simulink model "Bossi_Emanuele_EE460S3D_R99"  (R2025a)
settings: Solver=FixedStepDiscrete  StartTime=0.0  StopTime=120  FixedStep=dt0  RelTol=1e-3  EnableMultiTasking=on
PostLoadFcn:
  | %Set the size for the model
  | set_param(gcs,'Location',[10 10 1270 970])
  | %Set the zoom factor for the model
  | set_param(gcs,'ZoomFactor','100')
InitFcn:
  | tic
  | Bossi_Emanuele_EE460_Final
  | INIT_S3D_01
StartFcn:
  | tend0=toc;
  | tic;
StopFcn:
  | tend=toc;
  | disp(['Simulation time = ' num2str(tout(end)) ' sec'])
  | disp(['Real time = ' num2str(tend) ' sec'])
  | title('DONE')
  | SCORE=round((max(0,120-tout(end)-tend0))*4+10*(40-FuelBurned)+sum(100*double(PDONE)-100*double(PDONE<.5)));
  | PlotS3D(PlotInput);
  | text(15,22,['S: ' num2str(SCORE)]);
  | % Reset color scheme back to normal defaults
  | figure()
  | blkwhitebg('w');
  | close
values from neighbouring files (symbols this model uses):
  A_obs = [ 0  1  0  0  0  0 ... (first row only)    [Bossi_Emanuele_EE460_Final.m]
  B_obs = [ 0     0     0 ... (first row only)    [Bossi_Emanuele_EE460_Final.m]
  C_obs = [ 1 0 0 0 0 0 ... (first row only)    [Bossi_Emanuele_EE460_Final.m]
  d2r = pi/180    (= 0.0174532925199)    [INIT_S3D_01.m]
  D_obs = [ 0     0     0 ... (first row only)    [Bossi_Emanuele_EE460_Final.m]
  dt = 0.01    [INIT_S3D_01.m]
  dt0 = 0.001    [INIT_S3D_01.m]
  fr = 100    [INIT_S3D_01.m]
  G = [1,  1, -1, -1,  0,  0,  0,  0 ... (first row only)    [Bossi_Emanuele_EE460_Final.m]
  G_obs = eye(6)    [Bossi_Emanuele_EE460_Final.m]
  HM_S = 250    [INIT_S3D_01.m]
  HM_U = 500    [INIT_S3D_01.m]
  J = Jbase+JC0+JF+M*(Xcg^2+Ycg^2)    [INIT_S3D_01.m]
  Jbase = JC1+4*Ja+2*Ma*da^2+2*Ma*db^2    [INIT_S3D_01.m]
  JC0 = MC0/2    (= 10.2101761242)    [INIT_S3D_01.m]
  Kdtheta = 2 * zeta_th * wn_th * J_eff    [Bossi_Emanuele_EE460_Final.m]
  Kdtheta_fail = 2 * zeta_th_fail * wn_th_fail * J_eff    [Bossi_Emanuele_EE460_Final.m]
  Kdx = 2 * zeta_xy * wn_xy * M_eff    [Bossi_Emanuele_EE460_Final.m]
  Kdx_fail = 2 * zeta_xy_fail * wn_xy_fail * M_eff    [Bossi_Emanuele_EE460_Final.m]
  Kdy = 2 * zeta_xy * wn_xy * M_eff    [Bossi_Emanuele_EE460_Final.m]
  Kdy_fail = 2 * zeta_xy_fail * wn_xy_fail * M_eff    [Bossi_Emanuele_EE460_Final.m]
  Kptheta = J_eff * wn_th^2    [Bossi_Emanuele_EE460_Final.m]
  Kptheta_fail = J_eff * wn_th_fail^2    [Bossi_Emanuele_EE460_Final.m]
  Kpx = M_eff * wn_xy^2    [Bossi_Emanuele_EE460_Final.m]
  Kpx_fail = M_eff * wn_xy_fail^2    [Bossi_Emanuele_EE460_Final.m]
  Kpy = M_eff * wn_xy^2    [Bossi_Emanuele_EE460_Final.m]
  Kpy_fail = M_eff * wn_xy_fail^2    [Bossi_Emanuele_EE460_Final.m]
  L13 = sqrt(10)    [INIT_S3D_01.m]
  L24 = sqrt(6.25)    [INIT_S3D_01.m]
  LVL = LVL12    [INIT_S3D_01.m]
  M = MC+M1+M2+M3+M4+4*Ma    [INIT_S3D_01.m]
  M1 = LVL.M1    [INIT_S3D_01.m]
  M2 = LVL.M2    [INIT_S3D_01.m]
  M3 = LVL.M3    [INIT_S3D_01.m]
  M4 = LVL.M4    [INIT_S3D_01.m]
  max_qddot = [max_qddot_x; max_qddot_y; max_qddot_theta]    [Bossi_Emanuele_EE460_Final.m]
  mdti = (1/300)    (= 0.00333333333333)    [INIT_S3D_01.m]
  P = [1  1 -1 -1  0  0  0  0 ... (first row only)    [Bossi_Emanuele_EE460_Final.m]
  Pdata = [LVL.P1 LVL.P2 LVL.P3 LVL.P4]    [INIT_S3D_01.m]    (also in PlotS3D.m = R*[xt1;yt1+[0 3*tt*TV(idx-13)*TSIG(idx-13) 0]])
  PTvec = [Pdata(:,1);Pdata(:,2);Pdata(:,3);Pdata(:,4) ... (first row only)    [INIT_S3D_01.m]
  Q_obs = eye(6)    [Bossi_Emanuele_EE460_Final.m]
  r2d = 180/pi    (= 57.2957795131)    [INIT_S3D_01.m]
  r_bang = 0.5    [Bossi_Emanuele_EE460_Final.m]
  Sconfig = 1    [Bossi_Emanuele_EE460_Final.m]
  SLIM = [-100 100 ... (first row only)    [INIT_S3D_01.m]
  SQ = [.005 .01 .004 .005 .01 .004 .02 .01 .4]'    [INIT_S3D_01.m]
  SSF = 1./SQ    [INIT_S3D_01.m]
  tau = 0.5    [Bossi_Emanuele_EE460_Final.m]
  TOLdata = [LVL.P1tol LVL.P2tol LVL.P3tol LVL.P4tol]    [INIT_S3D_01.m]
  ULIM = [[Umin Umax];0 0;0 0]    [INIT_S3D_01.m]
undefined symbols (not defined in the file or in its folder): den_lp, den_lp2, DiscIntNeverNeededParam, dt1_bang_3, dt2_bang_3, dtc_bang_3, num_lp, num_lp2, q0_1
libraries: simulink x87, matrix_library x4, sl3dlib x1, aerolibutil x1, aerolibanimutils x1
(part 6 of 8)

== system Bossi_Emanuele_EE460S3D_R99/S3D_Plant/ThrusterValues/FailModes/Ufail4 ==
  Uin : Inport
  MP : Inport  Port=2
  Bus Selector1 : BusSelector  OutputSignals=U1cmd,U2cmd,U3cmd,U4cmd,U5cmd,U6cmd,U7cmd,U8cmd,U9cmd,U10cmd  OutputAsBus=on
  Bus Selector2 : BusSelector  OutputSignals=MfuelVector
  Bus to Vector2 : BusToVector
  CURRENT : Subsystem  TreatAsAtomicUnit=on
  Compare To Constant2 : simulink/Logic and Bit Operations/Compare To Constant  relop=>  const=eps  OutDataTypeStr=boolean
  Constant2 : Constant  Value=LVL.Uft(Udx,1)+rand*(LVL.Uft(Udx,2)-LVL.Uft(Udx,1))  SampleTime=dt0
  Constant3 : Constant  Value=LVL.Ufail(Udx)  SampleTime=dt0
  Constant4 : Constant  Value=-1  SampleTime=dt0
  Digital Clock : DigitalClock  SampleTime=dt0
  FailLogic : Subsystem
  If : If  IfExpression=u1 < -0.5  ElseIfExpressions=u1 > 0.5 & u1 < 1.5  SampleTime=dt0
  MAX : Subsystem  TreatAsAtomicUnit=on
  MIN : Subsystem  TreatAsAtomicUnit=on
  Merge : Merge  Inputs=3
  Relational Operator : RelationalOperator  Operator=<  OutDataTypeStr=boolean  InputSameDT=off
  Selector1 : Selector  InputPortWidth=4  IndexOptions=Index vector (dialog)  Indices=[Tank]  OutputSizes=1
  Selector2 : Selector  InputPortWidth=10  IndexOptions=Index vector (dialog)  Indices=[Udx]  OutputSizes=1
  Switch : Switch  Criteria=u2 > Threshold  SaturateOnIntegerOverflow=off  InputSameDT=off
  Switch1 : Switch  Criteria=u2 > Threshold  SaturateOnIntegerOverflow=off  InputSameDT=off
  Unit Delay : UnitDelay  SampleTime=dt0  HasFrameUpgradeWarning=on
  Uout : Outport
  wires:
  Selector2/1 -> Switch/1
  Bus to Vector2/1 -> Selector2/1
  Bus Selector1/1 -> Bus to Vector2/1
  FailLogic/1(NoFail) -> Switch/2
  Compare To Constant2/1 -> Switch1/2, FailLogic/2(FuelRemaining)
  Relational Operator/1 -> FailLogic/1(BeforeFail)
  Constant4/1 -> Switch1/3
  Constant3/1 -> Switch1/1
  Selector1/1 -> Compare To Constant2/1
  Bus Selector2/1 -> Selector1/1  "<MfuelVector>"
  MP/1 -> Bus Selector2/1
  Switch/1 -> Unit Delay/1, Uout/1
  Switch1/1 -> If/1, FailLogic/3(FailMode)
  Uin/1 -> Bus Selector1/1
  Merge/1 -> Switch/3
  MIN/1(Out1) -> Merge/1
  CURRENT/1(Out1) -> Merge/3
  Constant2/1 -> Relational Operator/2
  MAX/1(Out1) -> Merge/2
  Unit Delay/1 -> CURRENT/1(In1)
  If/3 -> CURRENT/Action
  Digital Clock/1 -> Relational Operator/1
  If/2 -> MAX/Action
  If/1 -> MIN/Action

== system Bossi_Emanuele_EE460S3D_R99/S3D_Plant/ThrusterValues/FailModes/Ufail5 ==
  Uin : Inport
  MP : Inport  Port=2
  Bus Selector1 : BusSelector  OutputSignals=U1cmd,U2cmd,U3cmd,U4cmd,U5cmd,U6cmd,U7cmd,U8cmd,U9cmd,U10cmd  OutputAsBus=on
  Bus Selector2 : BusSelector  OutputSignals=MfuelVector
  Bus to Vector2 : BusToVector
  CURRENT : Subsystem  TreatAsAtomicUnit=on
  Compare To Constant2 : simulink/Logic and Bit Operations/Compare To Constant  relop=>  const=eps  OutDataTypeStr=boolean
  Constant2 : Constant  Value=LVL.Uft(Udx,1)+rand*(LVL.Uft(Udx,2)-LVL.Uft(Udx,1))  SampleTime=dt0
  Constant3 : Constant  Value=LVL.Ufail(Udx)  SampleTime=dt0
  Constant4 : Constant  Value=-1  SampleTime=dt0
  Digital Clock : DigitalClock  SampleTime=dt0
  FailLogic : Subsystem
  If : If  IfExpression=u1 < -0.5  ElseIfExpressions=u1 > 0.5 & u1 < 1.5  SampleTime=dt0
  MAX : Subsystem  TreatAsAtomicUnit=on
  MIN : Subsystem  TreatAsAtomicUnit=on
  Merge : Merge  Inputs=3
  Relational Operator : RelationalOperator  Operator=<  OutDataTypeStr=boolean  InputSameDT=off
  Selector1 : Selector  InputPortWidth=4  IndexOptions=Index vector (dialog)  Indices=[Tank]  OutputSizes=1
  Selector2 : Selector  InputPortWidth=10  IndexOptions=Index vector (dialog)  Indices=[Udx]  OutputSizes=1
  Switch : Switch  Criteria=u2 > Threshold  SaturateOnIntegerOverflow=off  InputSameDT=off
  Switch1 : Switch  Criteria=u2 > Threshold  SaturateOnIntegerOverflow=off  InputSameDT=off
  Unit Delay : UnitDelay  SampleTime=dt0  HasFrameUpgradeWarning=on
  Uout : Outport
  wires:
  Selector2/1 -> Switch/1
  Bus to Vector2/1 -> Selector2/1
  Bus Selector1/1 -> Bus to Vector2/1
  FailLogic/1(NoFail) -> Switch/2
  Compare To Constant2/1 -> Switch1/2, FailLogic/2(FuelRemaining)
  Relational Operator/1 -> FailLogic/1(BeforeFail)
  Constant4/1 -> Switch1/3
  Constant3/1 -> Switch1/1
  Selector1/1 -> Compare To Constant2/1
  Bus Selector2/1 -> Selector1/1  "<MfuelVector>"
  MP/1 -> Bus Selector2/1
  Switch/1 -> Unit Delay/1, Uout/1
  Switch1/1 -> If/1, FailLogic/3(FailMode)
  Uin/1 -> Bus Selector1/1
  Merge/1 -> Switch/3
  MIN/1(Out1) -> Merge/1
  CURRENT/1(Out1) -> Merge/3
  Constant2/1 -> Relational Operator/2
  MAX/1(Out1) -> Merge/2
  Unit Delay/1 -> CURRENT/1(In1)
  If/3 -> CURRENT/Action
  Digital Clock/1 -> Relational Operator/1
  If/2 -> MAX/Action
  If/1 -> MIN/Action

== system Bossi_Emanuele_EE460S3D_R99/S3D_Plant/ThrusterValues/FailModes/Ufail6 ==
  Uin : Inport
  MP : Inport  Port=2
  Bus Selector1 : BusSelector  OutputSignals=U1cmd,U2cmd,U3cmd,U4cmd,U5cmd,U6cmd,U7cmd,U8cmd,U9cmd,U10cmd  OutputAsBus=on
  Bus Selector2 : BusSelector  OutputSignals=MfuelVector
  Bus to Vector2 : BusToVector
  CURRENT : Subsystem  TreatAsAtomicUnit=on
  Compare To Constant2 : simulink/Logic and Bit Operations/Compare To Constant  relop=>  const=eps  OutDataTypeStr=boolean
  Constant2 : Constant  Value=LVL.Uft(Udx,1)+rand*(LVL.Uft(Udx,2)-LVL.Uft(Udx,1))  SampleTime=dt0
  Constant3 : Constant  Value=LVL.Ufail(Udx)  SampleTime=dt0
  Constant4 : Constant  Value=-1  SampleTime=dt0
  Digital Clock : DigitalClock  SampleTime=dt0
  FailLogic : Subsystem
  If : If  IfExpression=u1 < -0.5  ElseIfExpressions=u1 > 0.5 & u1 < 1.5  SampleTime=dt0
  MAX : Subsystem  TreatAsAtomicUnit=on
  MIN : Subsystem  TreatAsAtomicUnit=on
  Merge : Merge  Inputs=3
  Relational Operator : RelationalOperator  Operator=<  OutDataTypeStr=boolean  InputSameDT=off
  Selector1 : Selector  InputPortWidth=4  IndexOptions=Index vector (dialog)  Indices=[Tank]  OutputSizes=1
  Selector2 : Selector  InputPortWidth=10  IndexOptions=Index vector (dialog)  Indices=[Udx]  OutputSizes=1
  Switch : Switch  Criteria=u2 > Threshold  SaturateOnIntegerOverflow=off  InputSameDT=off
  Switch1 : Switch  Criteria=u2 > Threshold  SaturateOnIntegerOverflow=off  InputSameDT=off
  Unit Delay : UnitDelay  SampleTime=dt0  HasFrameUpgradeWarning=on
  Uout : Outport
  wires:
  Selector2/1 -> Switch/1
  Bus to Vector2/1 -> Selector2/1
  Bus Selector1/1 -> Bus to Vector2/1
  FailLogic/1(NoFail) -> Switch/2
  Compare To Constant2/1 -> Switch1/2, FailLogic/2(FuelRemaining)
  Relational Operator/1 -> FailLogic/1(BeforeFail)
  Constant4/1 -> Switch1/3
  Constant3/1 -> Switch1/1
  Selector1/1 -> Compare To Constant2/1
  Bus Selector2/1 -> Selector1/1  "<MfuelVector>"
  MP/1 -> Bus Selector2/1
  Switch/1 -> Unit Delay/1, Uout/1
  Switch1/1 -> If/1, FailLogic/3(FailMode)
  Uin/1 -> Bus Selector1/1
  Merge/1 -> Switch/3
  MIN/1(Out1) -> Merge/1
  CURRENT/1(Out1) -> Merge/3
  Constant2/1 -> Relational Operator/2
  MAX/1(Out1) -> Merge/2
  Unit Delay/1 -> CURRENT/1(In1)
  If/3 -> CURRENT/Action
  Digital Clock/1 -> Relational Operator/1
  If/2 -> MAX/Action
  If/1 -> MIN/Action

== system Bossi_Emanuele_EE460S3D_R99/S3D_Plant/ThrusterValues/FailModes/Ufail7 ==
  Uin : Inport
  MP : Inport  Port=2
  Bus Selector1 : BusSelector  OutputSignals=U1cmd,U2cmd,U3cmd,U4cmd,U5cmd,U6cmd,U7cmd,U8cmd,U9cmd,U10cmd  OutputAsBus=on
  Bus Selector2 : BusSelector  OutputSignals=MfuelVector
  Bus to Vector2 : BusToVector
  CURRENT : Subsystem  TreatAsAtomicUnit=on
  Compare To Constant2 : simulink/Logic and Bit Operations/Compare To Constant  relop=>  const=eps  OutDataTypeStr=boolean
  Constant2 : Constant  Value=LVL.Uft(Udx,1)+rand*(LVL.Uft(Udx,2)-LVL.Uft(Udx,1))  SampleTime=dt0
  Constant3 : Constant  Value=LVL.Ufail(Udx)  SampleTime=dt0
  Constant4 : Constant  Value=-1  SampleTime=dt0
  Digital Clock : DigitalClock  SampleTime=dt0
  FailLogic : Subsystem
  If : If  IfExpression=u1 < -0.5  ElseIfExpressions=u1 > 0.5 & u1 < 1.5  SampleTime=dt0
  MAX : Subsystem  TreatAsAtomicUnit=on
  MIN : Subsystem  TreatAsAtomicUnit=on
  Merge : Merge  Inputs=3
  Relational Operator : RelationalOperator  Operator=<  OutDataTypeStr=boolean  InputSameDT=off
  Selector1 : Selector  InputPortWidth=4  IndexOptions=Index vector (dialog)  Indices=[Tank]  OutputSizes=1
  Selector2 : Selector  InputPortWidth=10  IndexOptions=Index vector (dialog)  Indices=[Udx]  OutputSizes=1
  Switch : Switch  Criteria=u2 > Threshold  SaturateOnIntegerOverflow=off  InputSameDT=off
  Switch1 : Switch  Criteria=u2 > Threshold  SaturateOnIntegerOverflow=off  InputSameDT=off
  Unit Delay : UnitDelay  SampleTime=dt0  HasFrameUpgradeWarning=on
  Uout : Outport
  wires:
  Selector2/1 -> Switch/1
  Bus to Vector2/1 -> Selector2/1
  Bus Selector1/1 -> Bus to Vector2/1
  FailLogic/1(NoFail) -> Switch/2
  Compare To Constant2/1 -> Switch1/2, FailLogic/2(FuelRemaining)
  Relational Operator/1 -> FailLogic/1(BeforeFail)
  Constant4/1 -> Switch1/3
  Constant3/1 -> Switch1/1
  Selector1/1 -> Compare To Constant2/1
  Bus Selector2/1 -> Selector1/1  "<MfuelVector>"
  MP/1 -> Bus Selector2/1
  Switch/1 -> Unit Delay/1, Uout/1
  Switch1/1 -> If/1, FailLogic/3(FailMode)
  Uin/1 -> Bus Selector1/1
  Merge/1 -> Switch/3
  MIN/1(Out1) -> Merge/1
  CURRENT/1(Out1) -> Merge/3
  Constant2/1 -> Relational Operator/2
  MAX/1(Out1) -> Merge/2
  Unit Delay/1 -> CURRENT/1(In1)
  If/3 -> CURRENT/Action
  Digital Clock/1 -> Relational Operator/1
  If/2 -> MAX/Action
  If/1 -> MIN/Action

== system Bossi_Emanuele_EE460S3D_R99/S3D_Plant/ThrusterValues/FailModes/Ufail8 ==
  Uin : Inport
  MP : Inport  Port=2
  Bus Selector1 : BusSelector  OutputSignals=U1cmd,U2cmd,U3cmd,U4cmd,U5cmd,U6cmd,U7cmd,U8cmd,U9cmd,U10cmd  OutputAsBus=on
  Bus Selector2 : BusSelector  OutputSignals=MfuelVector
  Bus to Vector2 : BusToVector
  CURRENT : Subsystem  TreatAsAtomicUnit=on
  Compare To Constant2 : simulink/Logic and Bit Operations/Compare To Constant  relop=>  const=eps  OutDataTypeStr=boolean
  Constant2 : Constant  Value=LVL.Uft(Udx,1)+rand*(LVL.Uft(Udx,2)-LVL.Uft(Udx,1))  SampleTime=dt0
  Constant3 : Constant  Value=LVL.Ufail(Udx)  SampleTime=dt0
  Constant4 : Constant  Value=-1  SampleTime=dt0
  Digital Clock : DigitalClock  SampleTime=dt0
  FailLogic : Subsystem
  If : If  IfExpression=u1 < -0.5  ElseIfExpressions=u1 > 0.5 & u1 < 1.5  SampleTime=dt0
  MAX : Subsystem  TreatAsAtomicUnit=on
  MIN : Subsystem  TreatAsAtomicUnit=on
  Merge : Merge  Inputs=3
  Relational Operator : RelationalOperator  Operator=<  OutDataTypeStr=boolean  InputSameDT=off
  Selector1 : Selector  InputPortWidth=4  IndexOptions=Index vector (dialog)  Indices=[Tank]  OutputSizes=1
  Selector2 : Selector  InputPortWidth=10  IndexOptions=Index vector (dialog)  Indices=[Udx]  OutputSizes=1
  Switch : Switch  Criteria=u2 > Threshold  SaturateOnIntegerOverflow=off  InputSameDT=off
  Switch1 : Switch  Criteria=u2 > Threshold  SaturateOnIntegerOverflow=off  InputSameDT=off
  Unit Delay : UnitDelay  SampleTime=dt0  HasFrameUpgradeWarning=on
  Uout : Outport
  wires:
  Selector2/1 -> Switch/1
  Bus to Vector2/1 -> Selector2/1
  Bus Selector1/1 -> Bus to Vector2/1
  FailLogic/1(NoFail) -> Switch/2
  Compare To Constant2/1 -> Switch1/2, FailLogic/2(FuelRemaining)
  Relational Operator/1 -> FailLogic/1(BeforeFail)
  Constant4/1 -> Switch1/3
  Constant3/1 -> Switch1/1
  Selector1/1 -> Compare To Constant2/1
  Bus Selector2/1 -> Selector1/1  "<MfuelVector>"
  MP/1 -> Bus Selector2/1
  Switch/1 -> Unit Delay/1, Uout/1
  Switch1/1 -> If/1, FailLogic/3(FailMode)
  Uin/1 -> Bus Selector1/1
  Merge/1 -> Switch/3
  MIN/1(Out1) -> Merge/1
  CURRENT/1(Out1) -> Merge/3
  Constant2/1 -> Relational Operator/2
  MAX/1(Out1) -> Merge/2
  Unit Delay/1 -> CURRENT/1(In1)
  If/3 -> CURRENT/Action
  Digital Clock/1 -> Relational Operator/1
  If/2 -> MAX/Action
  If/1 -> MIN/Action

== system Bossi_Emanuele_EE460S3D_R99/S3D_Plant/ThrusterValues/FailModes/Ufail9 ==
  Uin : Inport
  Bus Selector1 : BusSelector  OutputSignals=U1cmd,U2cmd,U3cmd,U4cmd,U5cmd,U6cmd,U7cmd,U8cmd,U9cmd,U10cmd  OutputAsBus=on
  Bus to Vector2 : BusToVector
  CURRENT : Subsystem  TreatAsAtomicUnit=on
  Constant2 : Constant  Value=LVL.Uft(Udx,1)+rand*(LVL.Uft(Udx,2)-LVL.Uft(Udx,1))  SampleTime=dt0
  Constant3 : Constant  Value=LVL.Ufail(Udx)  SampleTime=dt0
  Constant4 : Constant  Value=-1  SampleTime=dt0
  Constant5 : Constant  OutDataTypeStr=boolean  SampleTime=dt0
  Digital Clock : DigitalClock  SampleTime=dt0
  FailLogic : Subsystem
  If : If  IfExpression=u1 < -0.5  ElseIfExpressions=u1 > 0.5 & u1 < 1.5  SampleTime=dt0
  MAX : Subsystem  TreatAsAtomicUnit=on
  MIN : Subsystem  TreatAsAtomicUnit=on
  Merge : Merge  Inputs=3
  Relational Operator : RelationalOperator  Operator=<  OutDataTypeStr=boolean  InputSameDT=off
  Selector2 : Selector  InputPortWidth=10  IndexOptions=Index vector (dialog)  Indices=[Udx]  OutputSizes=1
  Switch : Switch  Criteria=u2 > Threshold  SaturateOnIntegerOverflow=off  InputSameDT=off
  Switch1 : Switch  Criteria=u2 > Threshold  SaturateOnIntegerOverflow=off  InputSameDT=off
  Unit Delay : UnitDelay  SampleTime=dt0  HasFrameUpgradeWarning=on
  Uout : Outport
  wires:
  Constant5/1 -> Switch1/2, FailLogic/2(FuelRemaining)
  Selector2/1 -> Switch/1
  Bus to Vector2/1 -> Selector2/1
  Bus Selector1/1 -> Bus to Vector2/1
  FailLogic/1(NoFail) -> Switch/2
  Relational Operator/1 -> FailLogic/1(BeforeFail)
  Constant4/1 -> Switch1/3
  Constant3/1 -> Switch1/1
  Switch/1 -> Unit Delay/1, Uout/1
  Switch1/1 -> If/1, FailLogic/3(FailMode)
  Uin/1 -> Bus Selector1/1
  Merge/1 -> Switch/3
  MIN/1(Out1) -> Merge/1
  CURRENT/1(Out1) -> Merge/3
  Constant2/1 -> Relational Operator/2
  MAX/1(Out1) -> Merge/2
  Unit Delay/1 -> CURRENT/1(In1)
  If/3 -> CURRENT/Action
  Digital Clock/1 -> Relational Operator/1
  If/2 -> MAX/Action
  If/1 -> MIN/Action

== system Bossi_Emanuele_EE460S3D_R99/S3D_Plant/ThrusterValues/HealthMonitoring/DetectFailures ==
  Uvalues : Inport
  UCMD : Inport  Port=2
  Bus Creator : BusCreator  Inputs=2
  Bus Creator1 : BusCreator  Inputs=10
  Bus Selector : BusSelector  OutputSignals=Ucmd.U1cmd,U.U1
  Bus Selector1 : BusSelector  OutputSignals=Ucmd.U2cmd,U.U2
  Bus Selector2 : BusSelector  OutputSignals=Ucmd.U3cmd,U.U3
  Bus Selector3 : BusSelector  OutputSignals=Ucmd.U4cmd,U.U4
  Bus Selector4 : BusSelector  OutputSignals=Ucmd.U5cmd,U.U5
  Bus Selector5 : BusSelector  OutputSignals=Ucmd.U6cmd,U.U6
  Bus Selector6 : BusSelector  OutputSignals=Ucmd.U7cmd,U.U7
  Bus Selector7 : BusSelector  OutputSignals=Ucmd.U8cmd,U.U8
  Bus Selector8 : BusSelector  OutputSignals=Ucmd.U9cmd,U.U9
  Bus Selector9 : BusSelector  OutputSignals=Ucmd.U10cmd,U.U10
  Subsystem : Subsystem
  Subsystem1 : Subsystem
  Subsystem2 : Subsystem
  Subsystem3 : Subsystem
  Subsystem4 : Subsystem
  Subsystem5 : Subsystem
  Subsystem6 : Subsystem
  Subsystem7 : Subsystem
  Subsystem8 : Subsystem
  Subsystem9 : Subsystem
  Out2 : Outport
  wires:
  Subsystem7/1(Out1) -> Bus Creator1/8  "U8fail"
  Bus Creator/1 -> Bus Selector/1, Bus Selector1/1, Bus Selector2/1, Bus Selector3/1, Bus Selector4/1, Bus Selector5/1, Bus Selector6/1, Bus Selector7/1, Bus Selector8/1, Bus Selector9/1
  Subsystem3/1(Out1) -> Bus Creator1/4  "U4fail"
  Subsystem9/1(Out1) -> Bus Creator1/10  "U10fail"
  Subsystem8/1(Out1) -> Bus Creator1/9  "U9fail"
  Subsystem1/1(Out1) -> Bus Creator1/2  "U2fail"
  Bus Selector9/2 -> Subsystem9/2(U)  "<U10>"
  Bus Selector1/1 -> Subsystem1/1(UCMD)  "<U2cmd>"
  Bus Selector8/1 -> Subsystem8/1(UCMD)  "<U9cmd>"
  Bus Selector1/2 -> Subsystem1/2(U)  "<U2>"
  Uvalues/1 -> Bus Creator/2
  Bus Selector6/2 -> Subsystem6/2(U)  "<U7>"
  Subsystem4/1(Out1) -> Bus Creator1/5  "U5fail"
  Bus Selector9/1 -> Subsystem9/1(UCMD)  "<U10cmd>"
  Bus Selector6/1 -> Subsystem6/1(UCMD)  "<U7cmd>"
  Subsystem2/1(Out1) -> Bus Creator1/3  "U3fail"
  Bus Selector3/1 -> Subsystem3/1(UCMD)  "<U4cmd>"
  Bus Selector5/2 -> Subsystem5/2(U)  "<U6>"
  Bus Selector7/1 -> Subsystem7/1(UCMD)  "<U8cmd>"
  Bus Selector8/2 -> Subsystem8/2(U)  "<U9>"
  Bus Selector4/1 -> Subsystem4/1(UCMD)  "<U5cmd>"
  Bus Creator1/1 -> Out2/1  "Ufail"
  Bus Selector5/1 -> Subsystem5/1(UCMD)  "<U6cmd>"
  Bus Selector2/2 -> Subsystem2/2(U)  "<U3>"
  Bus Selector4/2 -> Subsystem4/2(U)  "<U5>"
  Bus Selector3/2 -> Subsystem3/2(U)  "<U4>"
  Subsystem5/1(Out1) -> Bus Creator1/6  "U6fail"
  Bus Selector2/1 -> Subsystem2/1(UCMD)  "<U3cmd>"
  Bus Selector/1 -> Subsystem/1(UCMD)  "<U1cmd>"
  Bus Selector/2 -> Subsystem/2(U)  "<U1>"
  Subsystem6/1(Out1) -> Bus Creator1/7  "U7fail"
  Bus Selector7/2 -> Subsystem7/2(U)  "<U8>"
  Subsystem/1(Out1) -> Bus Creator1/1  "U1fail"
  UCMD/1 -> Bus Creator/1

== system Bossi_Emanuele_EE460S3D_R99/ControlLaw/Command/AutoMode/BangBang_cmd/InitialCondition ==
  In1 : Inport
  In2 : Inport  Port=2
  Relational Operator : RelationalOperator  Operator=~=  OutDataTypeStr=boolean  RndMeth=Simplest  InputSameDT=off
  Unit Delay : UnitDelay  SampleTime=dt  HasFrameUpgradeWarning=on
  Out1 : Outport
  Out2 : Outport  Port=2
  wires:
  In1/1 -> Out2/1
  In2/1 -> Unit Delay/1, Relational Operator/1
  Unit Delay/1 -> Relational Operator/2
  Relational Operator/1 -> Out1/1  "reset"

== system Bossi_Emanuele_EE460S3D_R99/ControlLaw/Command/AutoMode/BangBang_cmd/Precomputations ==
  CurrentPosition1 : Inport
  FinalPosition1 : Inport  Port=2
  CurrentVelocity : Inport  Port=3
  Bus Creator : BusCreator  Inputs=5
  ComputeBCBTimes : Subsystem
  Constant : Constant  Value=max_qddot  SampleTime=dt
  VariableTimer : Subsystem
  Out1 : Outport
  wires:
  Constant/1 -> ComputeBCBTimes/2(In2)
  ComputeBCBTimes/4(Acc) -> Bus Creator/5
  VariableTimer/1(Time_sec) -> Bus Creator/1
  ComputeBCBTimes/3(Out3) -> Bus Creator/4
  ComputeBCBTimes/1(Out4) -> VariableTimer/1(In1), Bus Creator/2  "TF_sec"
  CurrentPosition1/1 -> ComputeBCBTimes/1(CurrentPosition1)
  FinalPosition1/1 -> ComputeBCBTimes/3(FinalPosition1)
  ComputeBCBTimes/2(Out1) -> Bus Creator/3
  Bus Creator/1 -> Out1/1  "vars"
  CurrentVelocity/1 -> ComputeBCBTimes/4(CurrentVelocity)

== system Bossi_Emanuele_EE460S3D_R99/ControlLaw/Command/AutoMode/BangBang_cmd/ThetaTargetCorrector ==
  In2 : Inport
  In1 : Inport  Port=2
  AngleWrapper : Subsystem
  Mux : Mux  Inputs=3
  Selector : Selector  InputPortWidth=3  IndexOptions=Index vector (dialog)  Indices=[3]  OutputSizes=1
  Selector1 : Selector  InputPortWidth=3  IndexOptions=Index vector (dialog)  Indices=[3]  OutputSizes=1
  Selector2 : Selector  InputPortWidth=3  IndexOptions=Index vector (dialog)  Indices=[2]  OutputSizes=1
  Selector3 : Selector  InputPortWidth=3  IndexOptions=Index vector (dialog)  Indices=[1]  OutputSizes=1
  Sum : Sum  Inputs=|+-
  Sum1 : Sum  Inputs=|++
  Out1 : Outport
  wires:
  In2/1 -> Selector3/1, Selector2/1, Selector/1
  In1/1 -> Selector1/1
  Selector/1 -> Sum/1
  Selector1/1 -> Sum1/2, Sum/2
  Sum/1 -> AngleWrapper/1(In1)  "theta_deg"
  AngleWrapper/1(Out1) -> Sum1/1
  Sum1/1 -> Mux/3
  Mux/1 -> Out1/1
  Selector3/1 -> Mux/1
  Selector2/1 -> Mux/2

== system Bossi_Emanuele_EE460S3D_R99/ControlLaw/Command/AutoMode/FinalPositionSelector/Pdata1 ==
  Action Port : ActionPort  ActionPortLabel=if(u1 < 1.5)
  Constant : Constant  Value=Pdata(:, 1)  SampleTime=dt
  Out1 : Outport
  wires:
  Constant/1 -> Out1/1

== system Bossi_Emanuele_EE460S3D_R99/ControlLaw/Command/AutoMode/FinalPositionSelector/Pdata2 ==
  Action Port : ActionPort  ActionPortLabel=elseif(u1 < 2.5)
  Constant : Constant  Value=Pdata(:, 2)  SampleTime=dt
  Out1 : Outport
  wires:
  Constant/1 -> Out1/1

== system Bossi_Emanuele_EE460S3D_R99/ControlLaw/Command/AutoMode/FinalPositionSelector/Pdata3 ==
  Action Port : ActionPort  ActionPortLabel=elseif(u1 < 3.5)
  Constant : Constant  Value=Pdata(:, 3)  SampleTime=dt
  Out1 : Outport
  wires:
  Constant/1 -> Out1/1

== system Bossi_Emanuele_EE460S3D_R99/ControlLaw/Command/AutoMode/FinalPositionSelector/Pdata4 ==
  Action Port : ActionPort  ActionPortLabel=else
  Constant : Constant  Value=Pdata(:, 4)  SampleTime=dt
  Out1 : Outport
  wires:
  Constant/1 -> Out1/1

== system Bossi_Emanuele_EE460S3D_R99/ControlLaw/Command/InitialPoint/BangBang_cmd/Precomputations ==
  CurrentPosition1 : Inport
  Bus Creator : BusCreator  Inputs=5
  ComputeBCBTimes : Subsystem
  Constant : Constant  Value=max_qddot  SampleTime=dt
  VariableTimer : Subsystem
  Out1 : Outport
  wires:
  Constant/1 -> ComputeBCBTimes/2(In2)
  ComputeBCBTimes/4(Acc) -> Bus Creator/5
  VariableTimer/1(Time_sec) -> Bus Creator/1
  ComputeBCBTimes/3(Out3) -> Bus Creator/4
  ComputeBCBTimes/1(Out4) -> VariableTimer/1(In1), Bus Creator/2  "TF_sec"
  CurrentPosition1/1 -> ComputeBCBTimes/1(CurrentPosition1)
  ComputeBCBTimes/2(Out1) -> Bus Creator/3
  Bus Creator/1 -> Out1/1  "vars"

== system Bossi_Emanuele_EE460S3D_R99/ControlLaw/Command/InitialPoint/BangBang_cmd/ThetaTargetCorrector ==
  In2 : Inport
  In1 : Inport  Port=2
  AngleWrapper : Subsystem
  Mux : Mux  Inputs=3
  Selector : Selector  InputPortWidth=3  IndexOptions=Index vector (dialog)  Indices=[3]  OutputSizes=1
  Selector1 : Selector  InputPortWidth=3  IndexOptions=Index vector (dialog)  Indices=[3]  OutputSizes=1
  Selector2 : Selector  InputPortWidth=3  IndexOptions=Index vector (dialog)  Indices=[2]  OutputSizes=1
  Selector3 : Selector  InputPortWidth=3  IndexOptions=Index vector (dialog)  Indices=[1]  OutputSizes=1
  Sum : Sum  Inputs=|+-
  Sum1 : Sum  Inputs=|++
  Out1 : Outport
  wires:
  In2/1 -> Selector3/1, Selector2/1, Selector/1
  In1/1 -> Selector1/1
  Selector/1 -> Sum/1
  Selector1/1 -> Sum1/2, Sum/2
  Sum/1 -> AngleWrapper/1(In1)  "theta_deg"
  AngleWrapper/1(Out1) -> Sum1/1
  Sum1/1 -> Mux/3
  Mux/1 -> Out1/1
  Selector3/1 -> Mux/1
  Selector2/1 -> Mux/2

== system Bossi_Emanuele_EE460S3D_R99/ControlLaw/Command/Joystick/PointToGo/Hold ==
  In1 : Inport
  AND : Logic  IconShape=distinctive  AllPortsSameDT=off  OutDataTypeStr=boolean
  Bus Creator1 : BusCreator  Inputs=2
  Bus Selector1 : BusSelector  OutputSignals=MissionNum,UserChoice
  Bus Selector2 : BusSelector  OutputSignals=newSelection,MissionNumChanged
  Compare To Constant1 : simulink/Logic and Bit Operations/Compare To Constant  relop=>=  const=1.0  OutDataTypeStr=boolean
  Constant1 : Constant  Value=0
  Constant2 : Constant
  Relational Operator : RelationalOperator  Operator=~=  OutDataTypeStr=boolean  RndMeth=Simplest  InputSameDT=off
  Relational Operator1 : RelationalOperator  Operator=~=  OutDataTypeStr=boolean  RndMeth=Simplest  InputSameDT=off
  Switch : Switch  Criteria=u2 > Threshold  SaturateOnIntegerOverflow=off  InputSameDT=off
  Switch1 : Switch  Criteria=u2 > Threshold  SaturateOnIntegerOverflow=off  InputSameDT=off
  Unit Delay : UnitDelay  SampleTime=dt  HasFrameUpgradeWarning=on
  Unit Delay1 : UnitDelay  InitialCondition=1  SampleTime=dt  HasFrameUpgradeWarning=on
  Unit Delay2 : UnitDelay  SampleTime=dt  HasFrameUpgradeWarning=on
  Out1 : Outport
  Out2 : Outport  Port=2
  wires:
  Bus Creator1/1 -> Bus Selector2/1
  Bus Selector1/2 -> Compare To Constant1/1, Relational Operator1/1, Unit Delay/1  "<UserChoice>"
  Bus Selector2/1 -> Switch1/2  "<newSelection>"
  Bus Selector2/2 -> Switch/2  "<MissionNumChanged>"
  Unit Delay1/1 -> Relational Operator/2
  Bus Selector1/1 -> Relational Operator/1, Unit Delay1/1  "<MissionNum>"
  Switch1/1 -> Out1/1, Unit Delay2/1  "hold_active"
  Unit Delay2/1 -> Switch/3  "hold_prev"
  Compare To Constant1/1 -> AND/2
  Constant2/1 -> Switch1/1
  Relational Operator1/1 -> AND/1
  Switch/1 -> Switch1/3  "temp_hold"
  Constant1/1 -> Switch/1
  Unit Delay/1 -> Relational Operator1/2  "prev_UserChoice"
  Relational Operator/1 -> Bus Creator1/1  "MissionNumChanged"
  AND/1 -> Out2/1, Bus Creator1/2  "newSelection"
  In1/1 -> Bus Selector1/1

== system Bossi_Emanuele_EE460S3D_R99/ControlLaw/Observer/InternalObserver/L/ABM_INT3 ==
  DX : Inport
  Gain : Gain  Gain=23
  Gain1 : Gain  Gain=16
  Gain2 : Gain  Gain=5
  Product : Product  RndMeth=Zero
  Sum : Sum  Inputs=+-+
  Sum2 : Sum  Inputs=++|
  Unit Delay : UnitDelay  SampleTime=dt  HasFrameUpgradeWarning=on
  Unit Delay1 : UnitDelay  SampleTime=dt  HasFrameUpgradeWarning=on
  Unit Delay2 : UnitDelay  SampleTime=dt  HasFrameUpgradeWarning=on
  dt/12 : Constant  Value=dt/12  SampleTime=dt
  X : Outport
  wires:
  Sum2/1 -> Unit Delay/1
  Product/1 -> Sum2/2
  Unit Delay1/1 -> Gain1/1, Unit Delay2/1
  Gain/1 -> Sum/1
  Gain1/1 -> Sum/2
  Sum/1 -> Product/2
  DX/1 -> Gain/1, Unit Delay1/1
  Unit Delay/1 -> X/1, Sum2/1  "X"
  Gain2/1 -> Sum/3
  Unit Delay2/1 -> Gain2/1
  dt/12/1 -> Product/1

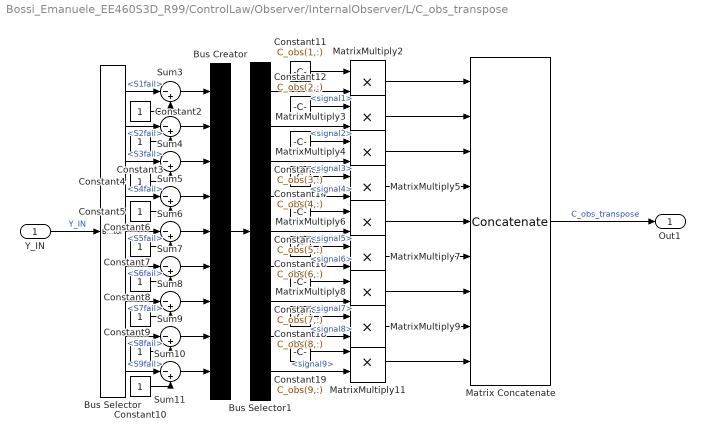
== system Bossi_Emanuele_EE460S3D_R99/ControlLaw/Observer/InternalObserver/L/C_obs_transpose ==
  Y_IN : Inport
  Bus Creator : BusCreator  Inputs=9
  Bus Selector : BusSelector  OutputSignals=S1fail,S2fail,S3fail,S4fail,S5fail,S6fail,S7fail,S8fail,S9fail
  Bus Selector1 : BusSelector  OutputSignals=signal1,signal2,signal3,signal4,signal5,signal6,signal7,signal8,signal9
  Constant{2..10} (9 alike) : Constant
  Constant11 : Constant  Value=C_obs(1,:)
  Constant12 : Constant  Value=C_obs(2,:)
  Constant13 : Constant  Value=C_obs(3,:)
  Constant14 : Constant  Value=C_obs(4,:)
  Constant15 : Constant  Value=C_obs(5,:)
  Constant16 : Constant  Value=C_obs(6,:)
  Constant17 : Constant  Value=C_obs(7,:)
  Constant18 : Constant  Value=C_obs(8,:)
  Constant19 : Constant  Value=C_obs(9,:)
  Matrix Concatenate : Concatenate  NumInputs=9  Mode=Multidimensional array  ConcatenateDimension=2
  MatrixMultiply{2..9,11} (9 alike) : Product
  Sum{3..11} (9 alike) : Sum  Inputs=|-+
  Out1 : Outport
  wires:
  Bus Selector1/3 -> MatrixMultiply4/2  "<signal3>"
  Constant12/1 -> MatrixMultiply3/1
  Constant3/1 -> Sum4/2
  Bus Selector1/4 -> MatrixMultiply5/2  "<signal4>"
  Bus Selector/8 -> Sum10/1  "<S8fail>"
  Constant17/1 -> MatrixMultiply8/1
  Constant16/1 -> MatrixMultiply7/1
  Bus Selector1/9 -> MatrixMultiply11/2  "<signal9>"
  Bus Selector1/1 -> MatrixMultiply2/2  "<signal1>"
  Bus Selector1/6 -> MatrixMultiply7/2  "<signal6>"
  Constant10/1 -> Sum11/2
  MatrixMultiply5/1 -> Matrix Concatenate/4
  Constant6/1 -> Sum7/2
  Bus Selector/3 -> Sum5/1  "<S3fail>"
  Sum6/1 -> Bus Creator/4
  Sum11/1 -> Bus Creator/9
  Bus Selector/7 -> Sum9/1  "<S7fail>"
  Sum4/1 -> Bus Creator/2
  Bus Selector/5 -> Sum7/1  "<S5fail>"
  Sum3/1 -> Bus Creator/1
  Bus Selector1/5 -> MatrixMultiply6/2  "<signal5>"
  MatrixMultiply6/1 -> Matrix Concatenate/5
  Constant11/1 -> MatrixMultiply2/1
  Constant18/1 -> MatrixMultiply9/1
  Constant8/1 -> Sum9/2
  MatrixMultiply9/1 -> Matrix Concatenate/8
  MatrixMultiply7/1 -> Matrix Concatenate/6
  Constant14/1 -> MatrixMultiply5/1
  Bus Selector/1 -> Sum3/1  "<S1fail>"
  Constant19/1 -> MatrixMultiply11/1
  MatrixMultiply8/1 -> Matrix Concatenate/7
  Constant5/1 -> Sum6/2
  Bus Selector/9 -> Sum11/1  "<S9fail>"
  Sum10/1 -> Bus Creator/8
  MatrixMultiply11/1 -> Matrix Concatenate/9
  Bus Creator/1 -> Bus Selector1/1
  Constant7/1 -> Sum8/2
  MatrixMultiply3/1 -> Matrix Concatenate/2
  Constant2/1 -> Sum3/2
  Constant9/1 -> Sum10/2
  Y_IN/1 -> Bus Selector/1  "Y_IN"
  Bus Selector/4 -> Sum6/1  "<S4fail>"
  Constant15/1 -> MatrixMultiply6/1
  Sum5/1 -> Bus Creator/3
  Sum7/1 -> Bus Creator/5
  Bus Selector1/8 -> MatrixMultiply9/2  "<signal8>"
  MatrixMultiply4/1 -> Matrix Concatenate/3
  Bus Selector1/2 -> MatrixMultiply3/2  "<signal2>"
  Bus Selector/6 -> Sum8/1  "<S6fail>"
  Constant13/1 -> MatrixMultiply4/1
  MatrixMultiply2/1 -> Matrix Concatenate/1
  Sum8/1 -> Bus Creator/6
  Sum9/1 -> Bus Creator/7
  Bus Selector/2 -> Sum4/1  "<S2fail>"
  Constant4/1 -> Sum5/2
  Bus Selector1/7 -> MatrixMultiply8/2  "<signal7>"
  Matrix Concatenate/1 -> Out1/1  "C_obs_transpose"

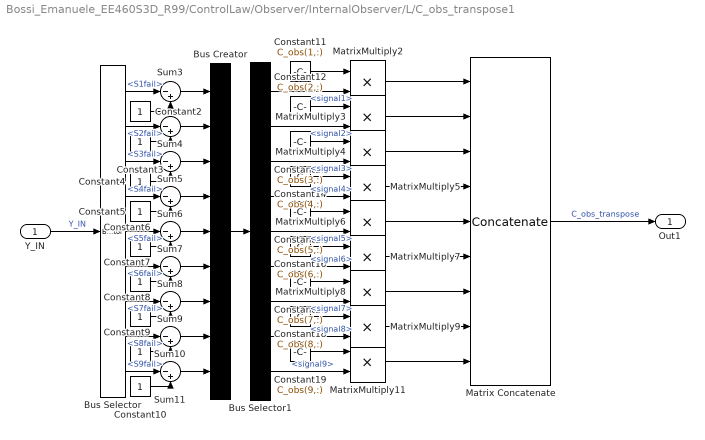
== system Bossi_Emanuele_EE460S3D_R99/ControlLaw/Observer/InternalObserver/L/C_obs_transpose1 ==
  Y_IN : Inport
  Bus Creator : BusCreator  Inputs=9
  Bus Selector : BusSelector  OutputSignals=S1fail,S2fail,S3fail,S4fail,S5fail,S6fail,S7fail,S8fail,S9fail
  Bus Selector1 : BusSelector  OutputSignals=signal1,signal2,signal3,signal4,signal5,signal6,signal7,signal8,signal9
  Constant{2..10} (9 alike) : Constant
  Constant11 : Constant  Value=C_obs(1,:)
  Constant12 : Constant  Value=C_obs(2,:)
  Constant13 : Constant  Value=C_obs(3,:)
  Constant14 : Constant  Value=C_obs(4,:)
  Constant15 : Constant  Value=C_obs(5,:)
  Constant16 : Constant  Value=C_obs(6,:)
  Constant17 : Constant  Value=C_obs(7,:)
  Constant18 : Constant  Value=C_obs(8,:)
  Constant19 : Constant  Value=C_obs(9,:)
  Matrix Concatenate : Concatenate  NumInputs=9  Mode=Multidimensional array  ConcatenateDimension=2
  MatrixMultiply{2..9,11} (9 alike) : Product
  Sum{3..11} (9 alike) : Sum  Inputs=|-+
  Out1 : Outport
  wires:
  Bus Selector1/3 -> MatrixMultiply4/2  "<signal3>"
  Constant12/1 -> MatrixMultiply3/1
  Constant3/1 -> Sum4/2
  Bus Selector1/4 -> MatrixMultiply5/2  "<signal4>"
  Bus Selector/8 -> Sum10/1  "<S8fail>"
  Constant17/1 -> MatrixMultiply8/1
  Constant16/1 -> MatrixMultiply7/1
  Bus Selector1/9 -> MatrixMultiply11/2  "<signal9>"
  Bus Selector1/1 -> MatrixMultiply2/2  "<signal1>"
  Bus Selector1/6 -> MatrixMultiply7/2  "<signal6>"
  Constant10/1 -> Sum11/2
  MatrixMultiply5/1 -> Matrix Concatenate/4
  Constant6/1 -> Sum7/2
  Bus Selector/3 -> Sum5/1  "<S3fail>"
  Sum6/1 -> Bus Creator/4
  Sum11/1 -> Bus Creator/9
  Bus Selector/7 -> Sum9/1  "<S7fail>"
  Sum4/1 -> Bus Creator/2
  Bus Selector/5 -> Sum7/1  "<S5fail>"
  Sum3/1 -> Bus Creator/1
  Bus Selector1/5 -> MatrixMultiply6/2  "<signal5>"
  MatrixMultiply6/1 -> Matrix Concatenate/5
  Constant11/1 -> MatrixMultiply2/1
  Constant18/1 -> MatrixMultiply9/1
  Constant8/1 -> Sum9/2
  MatrixMultiply9/1 -> Matrix Concatenate/8
  MatrixMultiply7/1 -> Matrix Concatenate/6
  Constant14/1 -> MatrixMultiply5/1
  Bus Selector/1 -> Sum3/1  "<S1fail>"
  Constant19/1 -> MatrixMultiply11/1
  MatrixMultiply8/1 -> Matrix Concatenate/7
  Constant5/1 -> Sum6/2
  Bus Selector/9 -> Sum11/1  "<S9fail>"
  Sum10/1 -> Bus Creator/8
  MatrixMultiply11/1 -> Matrix Concatenate/9
  Bus Creator/1 -> Bus Selector1/1
  Constant7/1 -> Sum8/2
  MatrixMultiply3/1 -> Matrix Concatenate/2
  Constant2/1 -> Sum3/2
  Constant9/1 -> Sum10/2
  Y_IN/1 -> Bus Selector/1  "Y_IN"
  Bus Selector/4 -> Sum6/1  "<S4fail>"
  Constant15/1 -> MatrixMultiply6/1
  Sum5/1 -> Bus Creator/3
  Sum7/1 -> Bus Creator/5
  Bus Selector1/8 -> MatrixMultiply9/2  "<signal8>"
  MatrixMultiply4/1 -> Matrix Concatenate/3
  Bus Selector1/2 -> MatrixMultiply3/2  "<signal2>"
  Bus Selector/6 -> Sum8/1  "<S6fail>"
  Constant13/1 -> MatrixMultiply4/1
  MatrixMultiply2/1 -> Matrix Concatenate/1
  Sum8/1 -> Bus Creator/6
  Sum9/1 -> Bus Creator/7
  Bus Selector/2 -> Sum4/1  "<S2fail>"
  Constant4/1 -> Sum5/2
  Bus Selector1/7 -> MatrixMultiply8/2  "<signal7>"
  Matrix Concatenate/1 -> Out1/1  "C_obs_transpose"

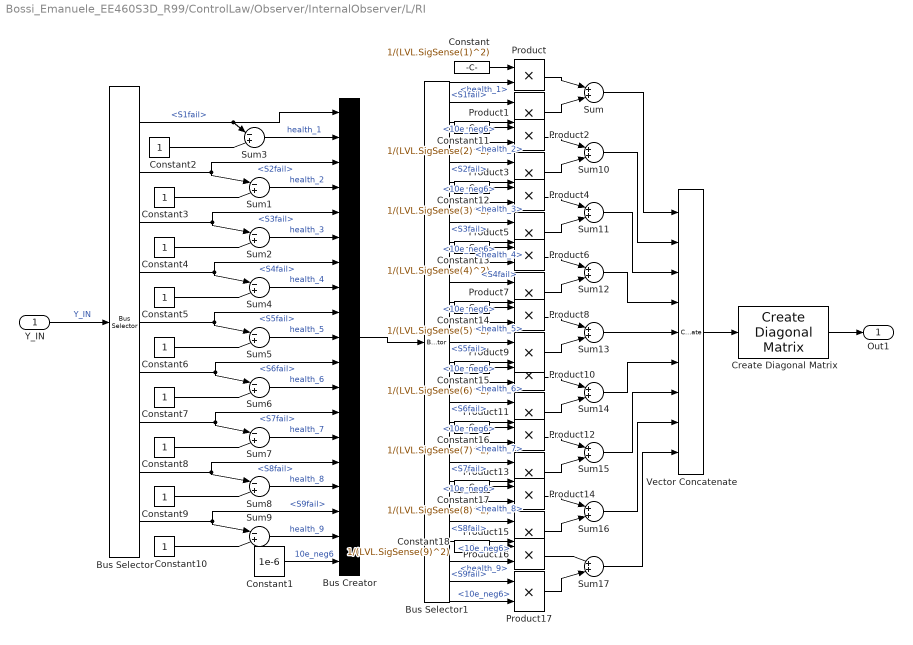
== system Bossi_Emanuele_EE460S3D_R99/ControlLaw/Observer/InternalObserver/L/RI ==
  Y_IN : Inport
  Bus Creator : BusCreator  Inputs=19
  Bus Selector : BusSelector  OutputSignals=S1fail,S2fail,S3fail,S4fail,S5fail,S6fail,S7fail,S8fail,S9fail
  Bus Selector1 : BusSelector  OutputSignals=health_1,S1fail,10e_neg6,health_2,S2fail,10e_neg6,health_3,S3fail,10e_neg6,health_4,S4fail,10e_neg6,health_5,S5fail,10e_neg6,health_6,S6fail,10e_neg6,health_7,S7fail,10e_neg6,health_8,S8fail,10e_neg6,health_9,S9fail,10e_neg6
  Constant : Constant  Value=1/(LVL.SigSense(1)^2)
  Constant1 : Constant  Value=1e-6
  Constant{2..10} (9 alike) : Constant
  Constant11 : Constant  Value=1/(LVL.SigSense(2)^2)
  Constant12 : Constant  Value=1/(LVL.SigSense(3)^2)
  Constant13 : Constant  Value=1/(LVL.SigSense(4)^2)
  Constant14 : Constant  Value=1/(LVL.SigSense(5)^2)
  Constant15 : Constant  Value=1/(LVL.SigSense(6)^2)
  Constant16 : Constant  Value=1/(LVL.SigSense(7)^2)
  Constant17 : Constant  Value=1/(LVL.SigSense(8)^2)
  Constant18 : Constant  Value=1/(LVL.SigSense(9)^2)
  Create Diagonal Matrix : matrix_library/Create Diagonal Matrix
      settings: LibrarySourceBlock=|
      | simulink/Matrix
      | Operations/Create Diagonal
      | Matrix
  Product{,1..17} (18 alike) : Product
  Sum{,10..17} (9 alike) : Sum  Inputs=|++|
  Sum{1..9} (9 alike) : Sum  Inputs=|-+|
  Vector Concatenate : Concatenate  NumInputs=9
  Out1 : Outport
  wires:
  Bus Selector/1 -> Bus Creator/1, Sum3/1  "<S1fail>"
  Y_IN/1 -> Bus Selector/1  "Y_IN"
  Constant2/1 -> Sum3/2
  Bus Creator/1 -> Bus Selector1/1
  Sum3/1 -> Bus Creator/2  "health_1"
  Constant3/1 -> Sum1/2
  Sum1/1 -> Bus Creator/4  "health_2"
  Constant4/1 -> Sum2/2
  Sum2/1 -> Bus Creator/6  "health_3"
  Constant5/1 -> Sum4/2
  Sum4/1 -> Bus Creator/8  "health_4"
  Constant6/1 -> Sum5/2
  Sum5/1 -> Bus Creator/10  "health_5"
  Constant7/1 -> Sum6/2
  Sum6/1 -> Bus Creator/12  "health_6"
  Constant8/1 -> Sum7/2
  Sum7/1 -> Bus Creator/14  "health_7"
  Constant9/1 -> Sum8/2
  Sum8/1 -> Bus Creator/16  "health_8"
  Constant10/1 -> Sum9/2
  Sum9/1 -> Bus Creator/18  "health_9"
  Bus Selector/2 -> Sum1/1, Bus Creator/3  "<S2fail>"
  Bus Selector/3 -> Sum2/1, Bus Creator/5  "<S3fail>"
  Bus Selector/4 -> Sum4/1, Bus Creator/7  "<S4fail>"
  Bus Selector/5 -> Sum5/1, Bus Creator/9  "<S5fail>"
  Bus Selector/6 -> Sum6/1, Bus Creator/11  "<S6fail>"
  Bus Selector/7 -> Sum7/1, Bus Creator/13  "<S7fail>"
  Bus Selector/8 -> Sum8/1, Bus Creator/15  "<S8fail>"
  Bus Selector/9 -> Sum9/1, Bus Creator/17  "<S9fail>"
  Constant1/1 -> Bus Creator/19  "10e_neg6"
  Constant/1 -> Product/1
  Bus Selector1/1 -> Product/2  "<health_1>"
  Bus Selector1/2 -> Product1/1  "<S1fail>"
  Bus Selector1/3 -> Product1/2  "<10e_neg6>"
  Product/1 -> Sum/1
  Product1/1 -> Sum/2
  Product3/1 -> Sum10/2
  Product2/1 -> Sum10/1
  Bus Selector1/4 -> Product2/2  "<health_2>"
  Bus Selector1/5 -> Product3/1  "<S2fail>"
  Bus Selector1/6 -> Product3/2  "<10e_neg6>"
  Product5/1 -> Sum11/2
  Product4/1 -> Sum11/1
  Bus Selector1/7 -> Product4/2  "<health_3>"
  Bus Selector1/8 -> Product5/1  "<S3fail>"
  Bus Selector1/9 -> Product5/2  "<10e_neg6>"
  Product7/1 -> Sum12/2
  Product6/1 -> Sum12/1
  Bus Selector1/11 -> Product7/1  "<S4fail>"
  Bus Selector1/12 -> Product7/2  "<10e_neg6>"
  Bus Selector1/10 -> Product6/2  "<health_4>"
  Product9/1 -> Sum13/2
  Product8/1 -> Sum13/1
  Bus Selector1/13 -> Product8/2  "<health_5>"
  Bus Selector1/14 -> Product9/1  "<S5fail>"
  Bus Selector1/15 -> Product9/2  "<10e_neg6>"
  Product11/1 -> Sum14/2
  Product10/1 -> Sum14/1
  Bus Selector1/16 -> Product10/2  "<health_6>"
  Bus Selector1/17 -> Product11/1  "<S6fail>"
  Bus Selector1/18 -> Product11/2  "<10e_neg6>"
  Product13/1 -> Sum15/2
  Product12/1 -> Sum15/1
  Bus Selector1/19 -> Product12/2  "<health_7>"
  Bus Selector1/20 -> Product13/1  "<S7fail>"
  Bus Selector1/21 -> Product13/2  "<10e_neg6>"
  Product15/1 -> Sum16/2
  Product14/1 -> Sum16/1
  Bus Selector1/22 -> Product14/2  "<health_8>"
  Bus Selector1/23 -> Product15/1  "<S8fail>"
  Bus Selector1/24 -> Product15/2  "<10e_neg6>"
  Product17/1 -> Sum17/2
  Product16/1 -> Sum17/1
  Bus Selector1/25 -> Product16/2  "<health_9>"
  Bus Selector1/27 -> Product17/2  "<10e_neg6>"
  Bus Selector1/26 -> Product17/1  "<S9fail>"
  Constant11/1 -> Product2/1
  Constant12/1 -> Product4/1
  Constant13/1 -> Product6/1
  Constant14/1 -> Product8/1
  Constant15/1 -> Product10/1
  Constant16/1 -> Product12/1
  Constant17/1 -> Product14/1
  Constant18/1 -> Product16/1
  Sum13/1 -> Vector Concatenate/5
  Sum14/1 -> Vector Concatenate/6
  Sum15/1 -> Vector Concatenate/7
  Sum16/1 -> Vector Concatenate/8
  Sum17/1 -> Vector Concatenate/9
  Sum12/1 -> Vector Concatenate/4
  Sum11/1 -> Vector Concatenate/3
  Sum10/1 -> Vector Concatenate/2
  Sum/1 -> Vector Concatenate/1
  Vector Concatenate/1 -> Create Diagonal Matrix/1
  Create Diagonal Matrix/1 -> Out1/1

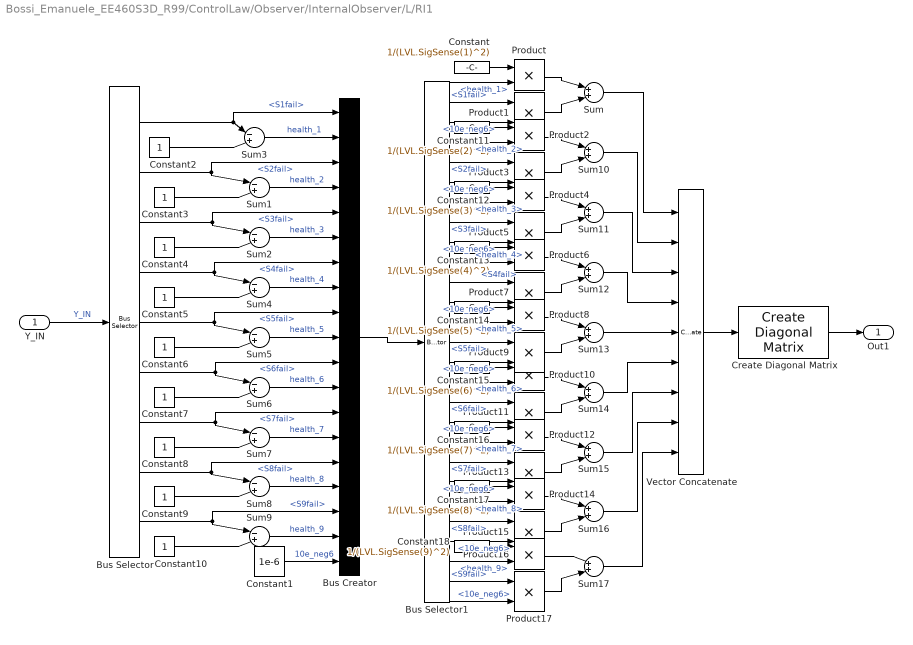
== system Bossi_Emanuele_EE460S3D_R99/ControlLaw/Observer/InternalObserver/L/RI1 ==
  Y_IN : Inport
  Bus Creator : BusCreator  Inputs=19
  Bus Selector : BusSelector  OutputSignals=S1fail,S2fail,S3fail,S4fail,S5fail,S6fail,S7fail,S8fail,S9fail
  Bus Selector1 : BusSelector  OutputSignals=health_1,S1fail,10e_neg6,health_2,S2fail,10e_neg6,health_3,S3fail,10e_neg6,health_4,S4fail,10e_neg6,health_5,S5fail,10e_neg6,health_6,S6fail,10e_neg6,health_7,S7fail,10e_neg6,health_8,S8fail,10e_neg6,health_9,S9fail,10e_neg6
  Constant : Constant  Value=1/(LVL.SigSense(1)^2)
  Constant1 : Constant  Value=1e-6
  Constant{2..10} (9 alike) : Constant
  Constant11 : Constant  Value=1/(LVL.SigSense(2)^2)
  Constant12 : Constant  Value=1/(LVL.SigSense(3)^2)
  Constant13 : Constant  Value=1/(LVL.SigSense(4)^2)
  Constant14 : Constant  Value=1/(LVL.SigSense(5)^2)
  Constant15 : Constant  Value=1/(LVL.SigSense(6)^2)
  Constant16 : Constant  Value=1/(LVL.SigSense(7)^2)
  Constant17 : Constant  Value=1/(LVL.SigSense(8)^2)
  Constant18 : Constant  Value=1/(LVL.SigSense(9)^2)
  Create Diagonal Matrix : matrix_library/Create Diagonal Matrix
      settings: LibrarySourceBlock=|
      | simulink/Matrix
      | Operations/Create Diagonal
      | Matrix
  Product{,1..17} (18 alike) : Product
  Sum{,10..17} (9 alike) : Sum  Inputs=|++|
  Sum{1..9} (9 alike) : Sum  Inputs=|-+|
  Vector Concatenate : Concatenate  NumInputs=9
  Out1 : Outport
  wires:
  Bus Selector/1 -> Bus Creator/1, Sum3/1  "<S1fail>"
  Y_IN/1 -> Bus Selector/1  "Y_IN"
  Constant2/1 -> Sum3/2
  Bus Creator/1 -> Bus Selector1/1
  Sum3/1 -> Bus Creator/2  "health_1"
  Constant3/1 -> Sum1/2
  Sum1/1 -> Bus Creator/4  "health_2"
  Constant4/1 -> Sum2/2
  Sum2/1 -> Bus Creator/6  "health_3"
  Constant5/1 -> Sum4/2
  Sum4/1 -> Bus Creator/8  "health_4"
  Constant6/1 -> Sum5/2
  Sum5/1 -> Bus Creator/10  "health_5"
  Constant7/1 -> Sum6/2
  Sum6/1 -> Bus Creator/12  "health_6"
  Constant8/1 -> Sum7/2
  Sum7/1 -> Bus Creator/14  "health_7"
  Constant9/1 -> Sum8/2
  Sum8/1 -> Bus Creator/16  "health_8"
  Constant10/1 -> Sum9/2
  Sum9/1 -> Bus Creator/18  "health_9"
  Bus Selector/2 -> Sum1/1, Bus Creator/3  "<S2fail>"
  Bus Selector/3 -> Sum2/1, Bus Creator/5  "<S3fail>"
  Bus Selector/4 -> Sum4/1, Bus Creator/7  "<S4fail>"
  Bus Selector/5 -> Sum5/1, Bus Creator/9  "<S5fail>"
  Bus Selector/6 -> Sum6/1, Bus Creator/11  "<S6fail>"
  Bus Selector/7 -> Sum7/1, Bus Creator/13  "<S7fail>"
  Bus Selector/8 -> Sum8/1, Bus Creator/15  "<S8fail>"
  Bus Selector/9 -> Sum9/1, Bus Creator/17  "<S9fail>"
  Constant1/1 -> Bus Creator/19  "10e_neg6"
  Constant/1 -> Product/1
  Bus Selector1/1 -> Product/2  "<health_1>"
  Bus Selector1/2 -> Product1/1  "<S1fail>"
  Bus Selector1/3 -> Product1/2  "<10e_neg6>"
  Product/1 -> Sum/1
  Product1/1 -> Sum/2
  Product3/1 -> Sum10/2
  Product2/1 -> Sum10/1
  Bus Selector1/4 -> Product2/2  "<health_2>"
  Bus Selector1/5 -> Product3/1  "<S2fail>"
  Bus Selector1/6 -> Product3/2  "<10e_neg6>"
  Product5/1 -> Sum11/2
  Product4/1 -> Sum11/1
  Bus Selector1/7 -> Product4/2  "<health_3>"
  Bus Selector1/8 -> Product5/1  "<S3fail>"
  Bus Selector1/9 -> Product5/2  "<10e_neg6>"
  Product7/1 -> Sum12/2
  Product6/1 -> Sum12/1
  Bus Selector1/11 -> Product7/1  "<S4fail>"
  Bus Selector1/12 -> Product7/2  "<10e_neg6>"
  Bus Selector1/10 -> Product6/2  "<health_4>"
  Product9/1 -> Sum13/2
  Product8/1 -> Sum13/1
  Bus Selector1/13 -> Product8/2  "<health_5>"
  Bus Selector1/14 -> Product9/1  "<S5fail>"
  Bus Selector1/15 -> Product9/2  "<10e_neg6>"
  Product11/1 -> Sum14/2
  Product10/1 -> Sum14/1
  Bus Selector1/16 -> Product10/2  "<health_6>"
  Bus Selector1/17 -> Product11/1  "<S6fail>"
  Bus Selector1/18 -> Product11/2  "<10e_neg6>"
  Product13/1 -> Sum15/2
  Product12/1 -> Sum15/1
  Bus Selector1/19 -> Product12/2  "<health_7>"
  Bus Selector1/20 -> Product13/1  "<S7fail>"
  Bus Selector1/21 -> Product13/2  "<10e_neg6>"
  Product15/1 -> Sum16/2
  Product14/1 -> Sum16/1
  Bus Selector1/22 -> Product14/2  "<health_8>"
  Bus Selector1/23 -> Product15/1  "<S8fail>"
  Bus Selector1/24 -> Product15/2  "<10e_neg6>"
  Product17/1 -> Sum17/2
  Product16/1 -> Sum17/1
  Bus Selector1/25 -> Product16/2  "<health_9>"
  Bus Selector1/27 -> Product17/2  "<10e_neg6>"
  Bus Selector1/26 -> Product17/1  "<S9fail>"
  Constant11/1 -> Product2/1
  Constant12/1 -> Product4/1
  Constant13/1 -> Product6/1
  Constant14/1 -> Product8/1
  Constant15/1 -> Product10/1
  Constant16/1 -> Product12/1
  Constant17/1 -> Product14/1
  Constant18/1 -> Product16/1
  Sum13/1 -> Vector Concatenate/5
  Sum14/1 -> Vector Concatenate/6
  Sum15/1 -> Vector Concatenate/7
  Sum16/1 -> Vector Concatenate/8
  Sum17/1 -> Vector Concatenate/9
  Sum12/1 -> Vector Concatenate/4
  Sum11/1 -> Vector Concatenate/3
  Sum10/1 -> Vector Concatenate/2
  Sum/1 -> Vector Concatenate/1
  Vector Concatenate/1 -> Create Diagonal Matrix/1
  Create Diagonal Matrix/1 -> Out1/1

== system Bossi_Emanuele_EE460S3D_R99/ControlLaw/Observer/SensorFailureHandling/Theta/ABM_INT2 ==
  DX : Inport
  Gain : Gain  Gain=23
  Gain1 : Gain  Gain=16
  Gain2 : Gain  Gain=5
  Product : Product  RndMeth=Zero
  Sum : Sum  Inputs=+-+
  Sum2 : Sum  Inputs=++|
  Unit Delay : UnitDelay  SampleTime=dt  HasFrameUpgradeWarning=on
  Unit Delay1 : UnitDelay  SampleTime=dt  HasFrameUpgradeWarning=on
  Unit Delay2 : UnitDelay  SampleTime=dt  HasFrameUpgradeWarning=on
  dt/12 : Constant  Value=dt/12  SampleTime=dt
  X : Outport
  wires:
  Sum2/1 -> Unit Delay/1
  Product/1 -> Sum2/2
  Unit Delay1/1 -> Gain1/1, Unit Delay2/1
  Gain/1 -> Sum/1
  Gain1/1 -> Sum/2
  Sum/1 -> Product/2
  DX/1 -> Gain/1, Unit Delay1/1
  Unit Delay/1 -> X/1, Sum2/1  "X"
  Gain2/1 -> Sum/3
  Unit Delay2/1 -> Gain2/1
  dt/12/1 -> Product/1

== system Bossi_Emanuele_EE460S3D_R99/ControlLaw/Observer/SensorFailureHandling/Theta/ABM_INT5 ==
  DX : Inport
  Gain : Gain  Gain=23
  Gain1 : Gain  Gain=16
  Gain2 : Gain  Gain=5
  Product : Product  RndMeth=Zero
  Sum : Sum  Inputs=+-+
  Sum2 : Sum  Inputs=++|
  Unit Delay : UnitDelay  SampleTime=dt  HasFrameUpgradeWarning=on
  Unit Delay1 : UnitDelay  SampleTime=dt  HasFrameUpgradeWarning=on
  Unit Delay2 : UnitDelay  SampleTime=dt  HasFrameUpgradeWarning=on
  dt/12 : Constant  Value=dt/12  SampleTime=dt
  X : Outport
  wires:
  Sum2/1 -> Unit Delay/1
  Product/1 -> Sum2/2
  Unit Delay1/1 -> Gain1/1, Unit Delay2/1
  Gain/1 -> Sum/1
  Gain1/1 -> Sum/2
  Sum/1 -> Product/2
  DX/1 -> Gain/1, Unit Delay1/1
  Unit Delay/1 -> X/1, Sum2/1  "X"
  Gain2/1 -> Sum/3
  Unit Delay2/1 -> Gain2/1
  dt/12/1 -> Product/1

== system Bossi_Emanuele_EE460S3D_R99/ControlLaw/Observer/SensorFailureHandling/X/ABM_INT ==
  DX : Inport
  Gain : Gain  Gain=23
  Gain1 : Gain  Gain=16
  Gain2 : Gain  Gain=5
  Product : Product  RndMeth=Zero
  Sum : Sum  Inputs=+-+
  Sum2 : Sum  Inputs=++|
  Unit Delay : UnitDelay  SampleTime=dt  HasFrameUpgradeWarning=on
  Unit Delay1 : UnitDelay  SampleTime=dt  HasFrameUpgradeWarning=on
  Unit Delay2 : UnitDelay  SampleTime=dt  HasFrameUpgradeWarning=on
  dt/12 : Constant  Value=dt/12  SampleTime=dt
  X : Outport
  wires:
  Sum2/1 -> Unit Delay/1
  Product/1 -> Sum2/2
  Unit Delay1/1 -> Gain1/1, Unit Delay2/1
  Gain/1 -> Sum/1
  Gain1/1 -> Sum/2
  Sum/1 -> Product/2
  DX/1 -> Gain/1, Unit Delay1/1
  Unit Delay/1 -> X/1, Sum2/1  "X"
  Gain2/1 -> Sum/3
  Unit Delay2/1 -> Gain2/1
  dt/12/1 -> Product/1

== system Bossi_Emanuele_EE460S3D_R99/ControlLaw/Observer/SensorFailureHandling/X/ABM_INT3 ==
  DX : Inport
  Gain : Gain  Gain=23
  Gain1 : Gain  Gain=16
  Gain2 : Gain  Gain=5
  Product : Product  RndMeth=Zero
  Sum : Sum  Inputs=+-+
  Sum2 : Sum  Inputs=++|
  Unit Delay : UnitDelay  SampleTime=dt  HasFrameUpgradeWarning=on
  Unit Delay1 : UnitDelay  SampleTime=dt  HasFrameUpgradeWarning=on
  Unit Delay2 : UnitDelay  SampleTime=dt  HasFrameUpgradeWarning=on
  dt/12 : Constant  Value=dt/12  SampleTime=dt
  X : Outport
  wires:
  Sum2/1 -> Unit Delay/1
  Product/1 -> Sum2/2
  Unit Delay1/1 -> Gain1/1, Unit Delay2/1
  Gain/1 -> Sum/1
  Gain1/1 -> Sum/2
  Sum/1 -> Product/2
  DX/1 -> Gain/1, Unit Delay1/1
  Unit Delay/1 -> X/1, Sum2/1  "X"
  Gain2/1 -> Sum/3
  Unit Delay2/1 -> Gain2/1
  dt/12/1 -> Product/1

== system Bossi_Emanuele_EE460S3D_R99/ControlLaw/Observer/SensorFailureHandling/Y/ABM_INT1 ==
  DX : Inport
  Gain : Gain  Gain=23
  Gain1 : Gain  Gain=16
  Gain2 : Gain  Gain=5
  Product : Product  RndMeth=Zero
  Sum : Sum  Inputs=+-+
  Sum2 : Sum  Inputs=++|
  Unit Delay : UnitDelay  SampleTime=dt  HasFrameUpgradeWarning=on
  Unit Delay1 : UnitDelay  SampleTime=dt  HasFrameUpgradeWarning=on
  Unit Delay2 : UnitDelay  SampleTime=dt  HasFrameUpgradeWarning=on
  dt/12 : Constant  Value=dt/12  SampleTime=dt
  X : Outport
  wires:
  Sum2/1 -> Unit Delay/1
  Product/1 -> Sum2/2
  Unit Delay1/1 -> Gain1/1, Unit Delay2/1
  Gain/1 -> Sum/1
  Gain1/1 -> Sum/2
  Sum/1 -> Product/2
  DX/1 -> Gain/1, Unit Delay1/1
  Unit Delay/1 -> X/1, Sum2/1  "X"
  Gain2/1 -> Sum/3
  Unit Delay2/1 -> Gain2/1
  dt/12/1 -> Product/1

== system Bossi_Emanuele_EE460S3D_R99/ControlLaw/Observer/SensorFailureHandling/Y/ABM_INT4 ==
  DX : Inport
  Gain : Gain  Gain=23
  Gain1 : Gain  Gain=16
  Gain2 : Gain  Gain=5
  Product : Product  RndMeth=Zero
  Sum : Sum  Inputs=+-+
  Sum2 : Sum  Inputs=++|
  Unit Delay : UnitDelay  SampleTime=dt  HasFrameUpgradeWarning=on
  Unit Delay1 : UnitDelay  SampleTime=dt  HasFrameUpgradeWarning=on
  Unit Delay2 : UnitDelay  SampleTime=dt  HasFrameUpgradeWarning=on
  dt/12 : Constant  Value=dt/12  SampleTime=dt
  X : Outport
  wires:
  Sum2/1 -> Unit Delay/1
  Product/1 -> Sum2/2
  Unit Delay1/1 -> Gain1/1, Unit Delay2/1
  Gain/1 -> Sum/1
  Gain1/1 -> Sum/2
  Sum/1 -> Product/2
  DX/1 -> Gain/1, Unit Delay1/1
  Unit Delay/1 -> X/1, Sum2/1  "X"
  Gain2/1 -> Sum/3
  Unit Delay2/1 -> Gain2/1
  dt/12/1 -> Product/1
